simulink model "Controle_da_Haste"  (R2025b)
settings: Solver=ode4  StartTime=0.0  StopTime=inf  FixedStep=0.01  RelTol=1e-3  EnableMultiTasking=on
undefined symbols (not defined in the file): bits
libraries: stm32blockslib x7
settings Model: STM32="{\"I2CControllerWrite\":[{\"ID\":\"untitled:10\"},{\"ID\":\"untitled:31\"},{\"ID\":\"untitled:32\"},{\"ID\":\"untitled:33\"},{\"ID\":\"Controle_da_Haste:31\"},{\"ID\":\"Controle_da_Haste:32\"},{\"ID\":\"Controle_da_Haste:33\"},{\"ID\":\"Controle_da_Haste:152\"},{\"ID\":\"Controle_da_Haste:153\"},{\"ID\":\"Controle_da_Haste:154\"},{\"ID\":\"Controle_da_Haste:10\"}],\"I2CControllerRead\":[{\"ID\":\"untitled:43\"},{\"ID\":\"Controle_da_Haste:43\"},{\"ID\":\"Controle_da_Haste:163\"}],\"EncoderBlock\":[{\"ID\":\"untitled:57\"},{\"ID\":\"Controle_da_Haste:57\"}],\"SPIControllerTransfer\":{\"ID\":\"Controle_da_Haste:81\"}}"  Creator=IEE-S  LastModifiedBy=IEE-S
settings OptimizationCC: EnhancedBackFolding=on  PassReuseOutputArgsAs=Individual arguments  ZeroExternalMemoryAtStartup=off  ZeroInternalMemoryAtStartup=off  MaxStackSize=512  OptimizeBlockOrder=speed  DifferentSizesBufferReuse=on  OptimizationCustomize=off  EfficientTunableParamExpr=on
settings DebuggingCC: ParameterTunabilityLossMsg=error
settings HardwareCC: ProdBitPerPointer=32.0  ProdBitPerSizeT=32.0  ProdBitPerPtrDiffT=32.0  ProdLargestAtomicInteger=Long  ProdLargestAtomicFloat=Double  ProdWordSize=32.0  ProdLongLongMode=on  ProdHWDeviceType=ARM Compatible->ARM Cortex-M
settings SFSimCC: MATLABDynamicMemAlloc=off
settings RTWCC: SystemTargetFile=ert.tlc  HardwareBoard=STM32F4xx Based  TemplateMakefile=ert_default_tmf  Toolchain=GNU Tools for ARM Embedded Processors  Description=Embedded Coder
settings CodeAppCC: ForceParamTrailComments=on  IgnoreCustomStorageClasses=off  OperatorAnnotations=on  SimulinkDataObjDesc=on  SFDataObjDesc=on  InsertBlockDesc=on
settings ERTTargetCC: ExtModeTransport=3.0  ExtModeStaticAlloc=on  ExtModeStaticAllocSize=2048.0  ExtModeMexFile=ext_xcp  ExtModeIntrfLevel=Level2 - Open  InlinedParameterPlacement=Hierarchical  TargetLangStandard=C99 (ISO)  CodeReplacementLibrary=ARM Cortex-M

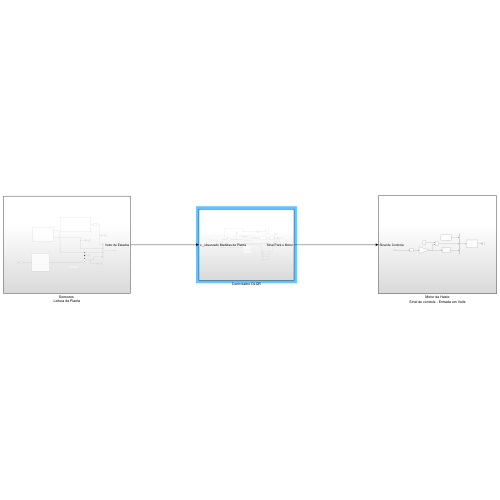
[thumbnail: Simulink's stored preview of the top-level diagram]
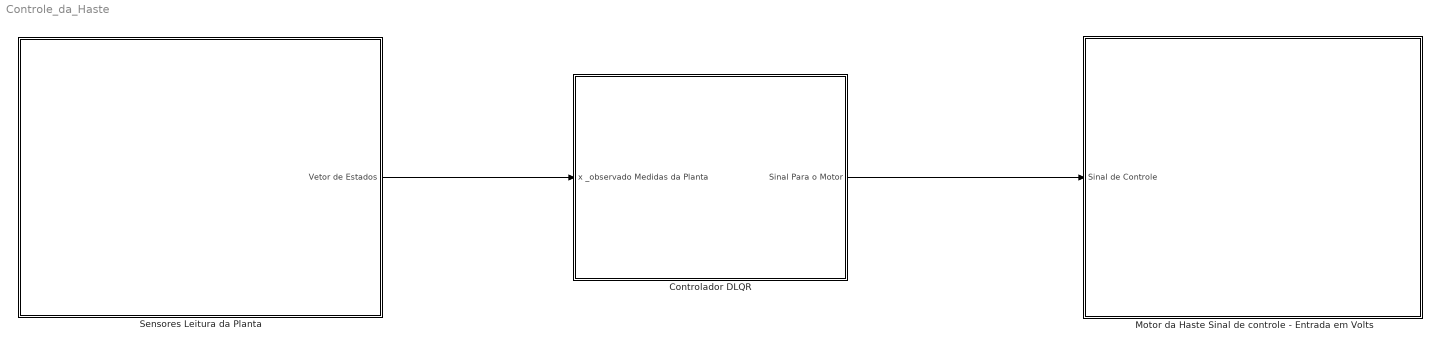
== system Controle_da_Haste ==
  Controlador DLQR : Subsystem
  Motor da Haste Sinal de controle - Entrada em Volts : Subsystem  Priority=6
  Sensores Leitura da Planta : Subsystem
  wires:
  Sensores Leitura da Planta/1(Vetor de Estados) -> Controlador DLQR/1(x _observado Medidas da Planta)
  Controlador DLQR/1(Sinal Para o Motor) -> Motor da Haste Sinal de controle - Entrada em Volts/1(Sinal de Controle)

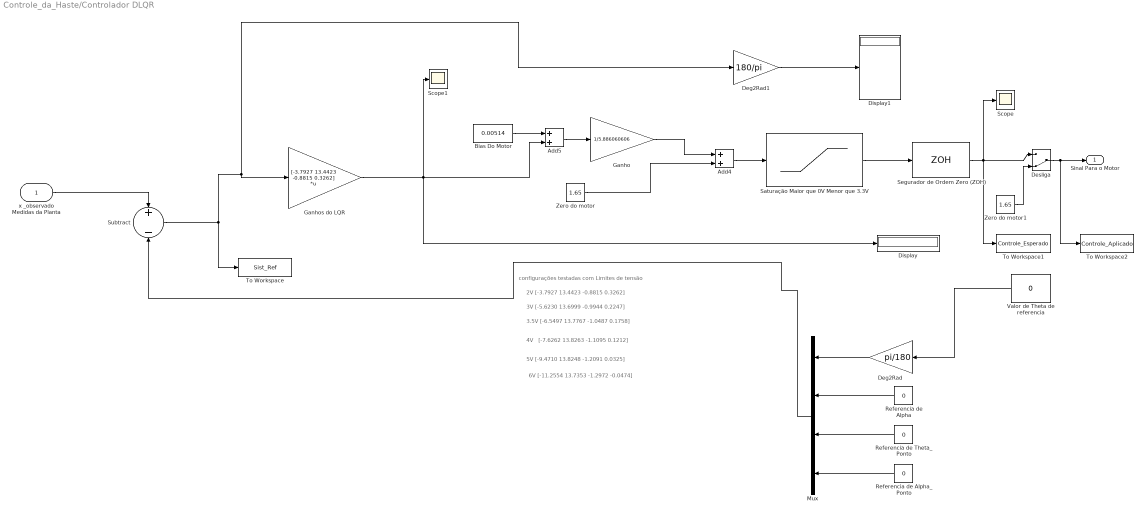
== system Controle_da_Haste/Controlador DLQR ==
  note: [-7.6262 13.8263 -1.1095 0.1212]
  note: 4V
  note: 3V [-5.6230 13.6999 -0.9944 0.2247]
  note: 2V [-3.7927 13.4423 -0.8815 0.3262]
  note: configurações testadas com Limites de tensão
  note: 3.5V [-6.5497 13.7767 -1.0487 0.1758]
  note: 5V [-9.4710 13.8248 -1.2091 0.0325]
  note: 6V [-11.2554 13.7353 -1.2972 -0.0474]
  x _observado Medidas da Planta : Inport
  Add4 : Sum
  Add5 : Sum
  Bias Do Motor : Constant  Value=0.00514
  Deg2Rad : Gain  Gain=pi/180
  Deg2Rad1 : Gain  Gain=180/pi
  Desliga : ManualSwitch  CurrentSetting=0
  Display : Display
  Display1 : Display
  Ganho : Gain  Gain=1/5.886060606
  Ganhos do LQR : Gain  Gain="[-3.7927  13.4423    -0.8815   0.3262]"  Multiplication=Matrix(K*u) (u vector)
  Mux : Mux
  Referencia de Alpha : Constant  Value=0
  Referencia de Alpha_Ponto : Constant  Value=0
  Referencia de Theta_Ponto : Constant  Value=0
  Saturação Maior que 0V Menor que 3.3V : Saturate  UpperLimit=3.3  LowerLimit=0
  Scope : Scope
      settings: ActiveDisplayYMinimum=1.3696990193816192  ActiveDisplayYMaximum=1.8844669389329192  DataLoggingVariableName=ScopeData4
  Scope1 : Scope
      settings: ActiveDisplayYMinimum=-26.689119690198989  ActiveDisplayYMaximum=29.989428485909986  DataLoggingVariableName=ScopeData5
  Segurador de Ordem Zero (ZOH) : ZeroOrderHold  SampleTime=-1
  Subtract : Sum  Inputs=+-
  To Workspace : ToWorkspace  VariableName=Sist_Ref  SaveFormat=Timeseries  SampleTime=-1
  To Workspace1 : ToWorkspace  VariableName=Controle_Esperado  SaveFormat=Timeseries  SampleTime=-1
  To Workspace2 : ToWorkspace  VariableName=Controle_Aplicado  SaveFormat=Timeseries  SampleTime=-1
  Valor de Theta de referencia : Constant  Value=0
  Zero do motor : Constant  Value=1.65
  Zero do motor1 : Constant  Value=1.65
  Sinal Para o Motor : Outport
  wires:
  x _observado Medidas da Planta/1 -> Subtract/1
  Bias Do Motor/1 -> Add5/1
  Ganho/1 -> Add4/1
  Zero do motor/1 -> Add4/2
  Add4/1 -> Saturação Maior que 0V Menor que 3.3V/1
  Add5/1 -> Ganho/1
  Ganhos do LQR/1 -> Scope1/1, Add5/2, Display/1
  Saturação Maior que 0V Menor que 3.3V/1 -> Segurador de Ordem Zero (ZOH)/1
  Subtract/1 -> To Workspace/1, Deg2Rad1/1, Ganhos do LQR/1
  Segurador de Ordem Zero (ZOH)/1 -> Scope/1, Desliga/1, To Workspace1/1
  Deg2Rad/1 -> Mux/1
  Referencia de Theta_Ponto/1 -> Mux/3
  Referencia de Alpha/1 -> Mux/2
  Referencia de Alpha_Ponto/1 -> Mux/4
  Mux/1 -> Subtract/2
  Desliga/1 -> To Workspace2/1, Sinal Para o Motor/1
  Zero do motor1/1 -> Desliga/2
  Valor de Theta de referencia/1 -> Deg2Rad/1
  Deg2Rad1/1 -> Display1/1

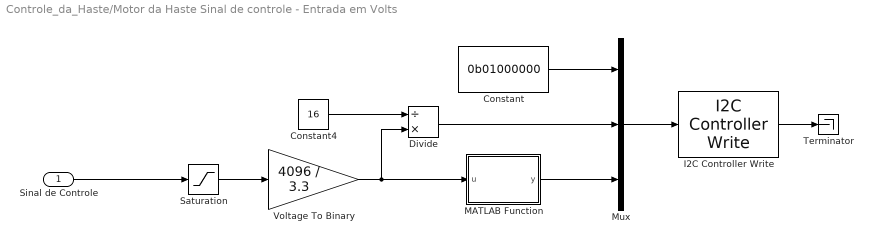
== system Controle_da_Haste/Motor da Haste Sinal de controle - Entrada em Volts ==
  Sinal de Controle : Inport
  Constant : Constant  Value=0b01000000  OutDataTypeStr=uint8
  Constant4 : Constant  Value=16
  Divide : Product  Inputs=/*  OutDataTypeStr=uint8
  I2C Controller Write : stm32blockslib/I2C Controller Write  I2CModule=I2C1  Mode=Controller  AddressingMode=7-bits  PeripheralByteOrder=BigEndian  OwnPeripheralAddress=uint8(170)  PeripheralAddressVia=Dialog  PeripheralAddress=0x60  RegisterAddressMode=off  RegisterAddressVia=Dialog  RegisterAddress=1  RepeatedStart=off  NoAck=off  OutputStatus=on  BlockMode=Transmit  DataType=uint8  DataLength=1  Timeout=0.001  SampleTime=-1
      settings: LibrarySourceBlock=stm32f4xxblockslib/I2C Controller Write
  MATLAB Function : MATLAB Function  TreatAsAtomicUnit=on
  Mux : Mux  Inputs=3
  Saturation : Saturate  UpperLimit=3.3  LowerLimit=0  OutDataTypeStr=Inherit: Inherit via back propagation
  Terminator : Terminator
  Voltage To Binary : Gain  Gain=4096 / 3.3  ParamDataTypeStr=uint16
  wires:
  Voltage To Binary/1 -> Divide/2, MATLAB Function/1(u)
  Constant4/1 -> Divide/1
  Constant/1 -> Mux/1
  Divide/1 -> Mux/2
  I2C Controller Write/1 -> Terminator/1
  MATLAB Function/1(y) -> Mux/3
  Saturation/1 -> Voltage To Binary/1
  Mux/1 -> I2C Controller Write/1
  Sinal de Controle/1 -> Saturation/1

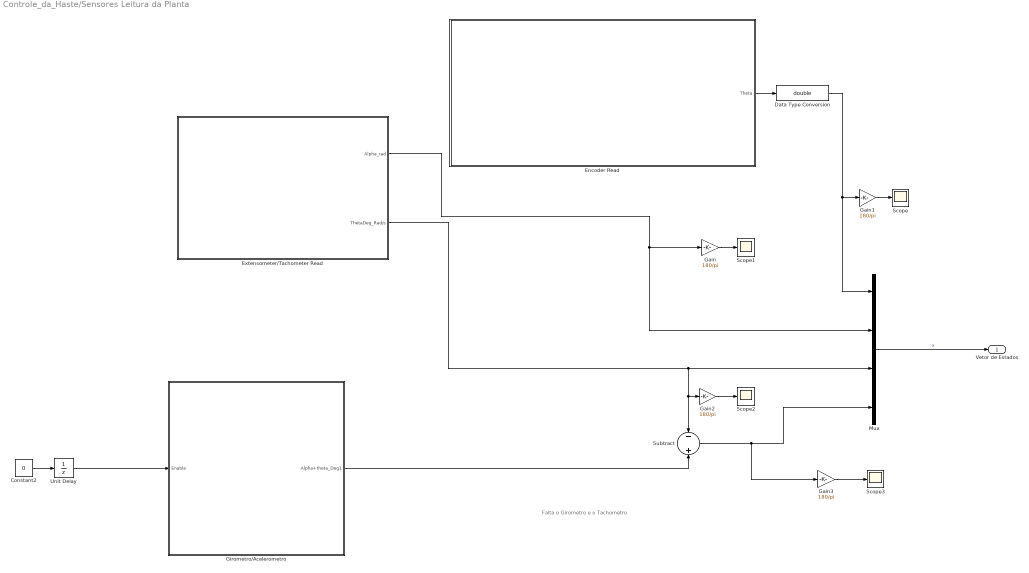
== system Controle_da_Haste/Sensores Leitura da Planta ==
  note: Falta o Girometro e o Tachometro
  Constant2 : Constant  Value=0
  Data Type Conversion : DataTypeConversion  OutDataTypeStr=double  RndMeth=Round  SaturateOnIntegerOverflow=off
  Encoder Read : Subsystem  Priority=3
  Extensometer/Tachometer Read : Subsystem  Priority=4
  Gain{,1..3} (4 alike) : Gain  Gain=180/pi
  Girometro/Acelerometro : Subsystem  Priority=1
  Mux : Mux
  Scope{,1..3} (4 alike) : Scope
      Scope settings: ActiveDisplayYMinimum=-37.614862788092672  ActiveDisplayYMaximum=73.168879201509782
      Scope1 settings: ActiveDisplayYMinimum=-4.0610934597852637  ActiveDisplayYMaximum=0.45969850920646227
      Scope2 settings: ActiveDisplayYMinimum=-2.80662625539894  ActiveDisplayYMaximum=8.42656069865145  DataLoggingVariableName=ScopeData2
      Scope3 settings: ActiveDisplayYMinimum=-35.050597654455132  ActiveDisplayYMaximum=20.146961930229978  DataLoggingVariableName=ScopeData3
  Subtract : Sum  Inputs=-+
  Unit Delay : UnitDelay  InitialCondition=1  SampleTime=-1  HasFrameUpgradeWarning=on
  Vetor de Estados : Outport
  wires:
  Mux/1 -> Vetor de Estados/1  "x"
  Extensometer/Tachometer Read/2(ThetaDeg_Rad/s) -> Gain2/1, Subtract/1, Mux/3
  Encoder Read/1(Theta) -> Data Type Conversion/1
  Subtract/1 -> Mux/4, Gain3/1
  Girometro/Acelerometro/1(Alpha+theta_Deg1) -> Subtract/2
  Unit Delay/1 -> Girometro/Acelerometro/1(Enable)
  Constant2/1 -> Unit Delay/1
  Extensometer/Tachometer Read/1(Alpha_rad) -> Mux/2, Gain/1
  Data Type Conversion/1 -> Gain1/1, Mux/1
  Gain/1 -> Scope1/1
  Gain1/1 -> Scope/1
  Gain2/1 -> Scope2/1
  Gain3/1 -> Scope3/1

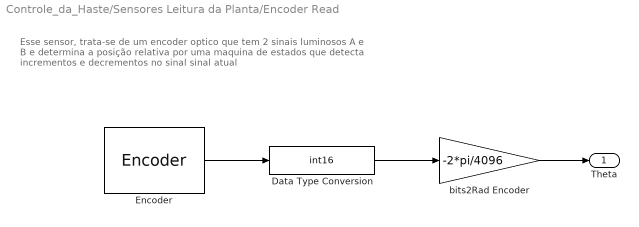
== system Controle_da_Haste/Sensores Leitura da Planta/Encoder Read ==
  note: Esse sensor, trata-se de um encoder optico que tem 2 sinais luminosos A e B e determina a posição relativa por uma maquina de estados que detecta incrementos e decrementos no sinal sinal atual
  Data Type Conversion : DataTypeConversion  OutDataTypeStr=int16  RndMeth=Round  SaturateOnIntegerOverflow=off
  Encoder : stm32blockslib/Encoder  TimerModule=TIM4  EnableResetInput=off  OutputDirection=off  SampleTime=-1
      settings: LibrarySourceBlock=stm32f4xxblockslib/Encoder
  bits2Rad Encoder : Gain  Gain=-2*pi/4096
  Theta : Outport
  wires:
  Encoder/1 -> Data Type Conversion/1
  Data Type Conversion/1 -> bits2Rad Encoder/1
  bits2Rad Encoder/1 -> Theta/1

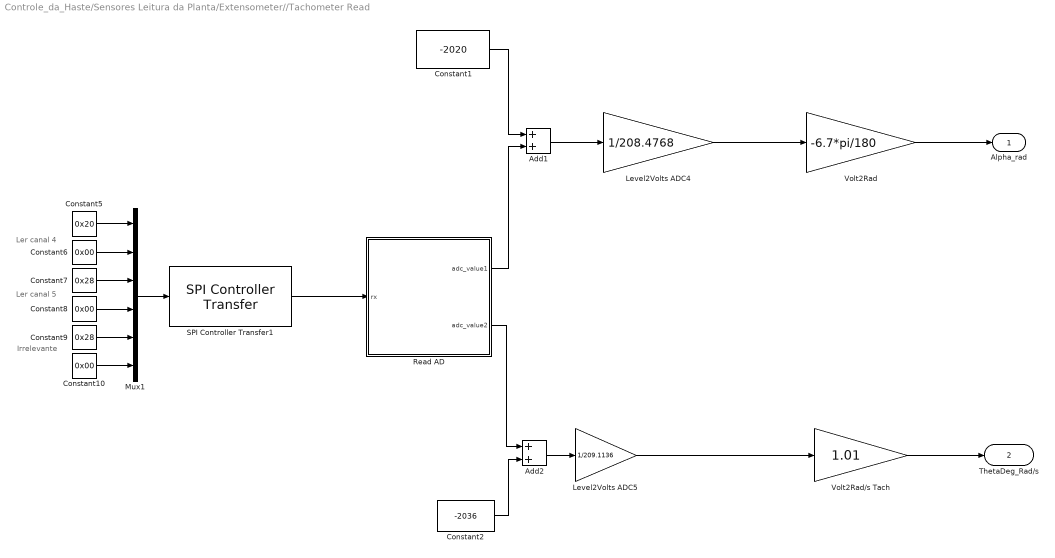
== system Controle_da_Haste/Sensores Leitura da Planta/Extensometer//Tachometer Read ==
  note: Irrelevante
  note: Ler canal 5
  note: Ler canal 4
  Add1 : Sum
  Add2 : Sum
  Constant1 : Constant  Value=-2020
  Constant10 : Constant  Value=0x00  OutDataTypeStr=uint8
  Constant2 : Constant  Value=-2036
  Constant5 : Constant  Value=0x20  OutDataTypeStr=uint8
  Constant6 : Constant  Value=0x00  OutDataTypeStr=uint8
  Constant7 : Constant  Value=0x28  OutDataTypeStr=uint8
  Constant8 : Constant  Value=0x00  OutDataTypeStr=uint8
  Constant9 : Constant  Value=0x28  OutDataTypeStr=uint8
  Level2Volts ADC4 : Gain  Gain=1/208.4768
  Level2Volts ADC5 : Gain  Gain=1/209.1136
  Mux1 : Mux  Inputs=6
  Read AD : MATLAB Function  TreatAsAtomicUnit=on
  SPI Controller Transfer1 : stm32blockslib/SPI Controller Transfer  SPIModuleSelect=SPI2  ClockPolarity=Low  ClockPhase=1 Edge  SPIModule=uint32(0)  Mode=Master  BusSpeed=uint32(1000000)  FirstBitToTransfer=Most significant bit (MSB)  ClockMode=0  BlockFunction=Transfer  EnableRegisterAddress=off  RegisterAddress=0  OutputDataType=uint8  OutputDataLength=1  OutputStatus=off  BlockingMode=on  Timeout=1  DataBits=8  UseCustomSSPin=Explicit GPIO calls  ActiveLowSSPin=Active low  Port_Select=GPIOA  Pin=4
      settings: LibrarySourceBlock=stm32f4xxblockslib/SPI Controller Transfer
  Volt2Rad : Gain  Gain=-6.7*pi/180
  Volt2Rad/s Tach : Gain  Gain=1.01
  Alpha_rad : Outport
  ThetaDeg_Rad/s : Outport  Port=2
  wires:
  Constant8/1 -> Mux1/4
  Constant7/1 -> Mux1/3
  Constant5/1 -> Mux1/1
  Mux1/1 -> SPI Controller Transfer1/1
  SPI Controller Transfer1/1 -> Read AD/1(rx)
  Constant6/1 -> Mux1/2
  Constant10/1 -> Mux1/6
  Constant9/1 -> Mux1/5
  Level2Volts ADC5/1 -> Volt2Rad/s Tach/1
  Level2Volts ADC4/1 -> Volt2Rad/1
  Volt2Rad/s Tach/1 -> ThetaDeg_Rad/s/1
  Volt2Rad/1 -> Alpha_rad/1
  Add1/1 -> Level2Volts ADC4/1
  Read AD/1(adc_value1) -> Add1/2
  Constant1/1 -> Add1/1
  Add2/1 -> Level2Volts ADC5/1
  Read AD/2(adc_value2) -> Add2/1
  Constant2/1 -> Add2/2

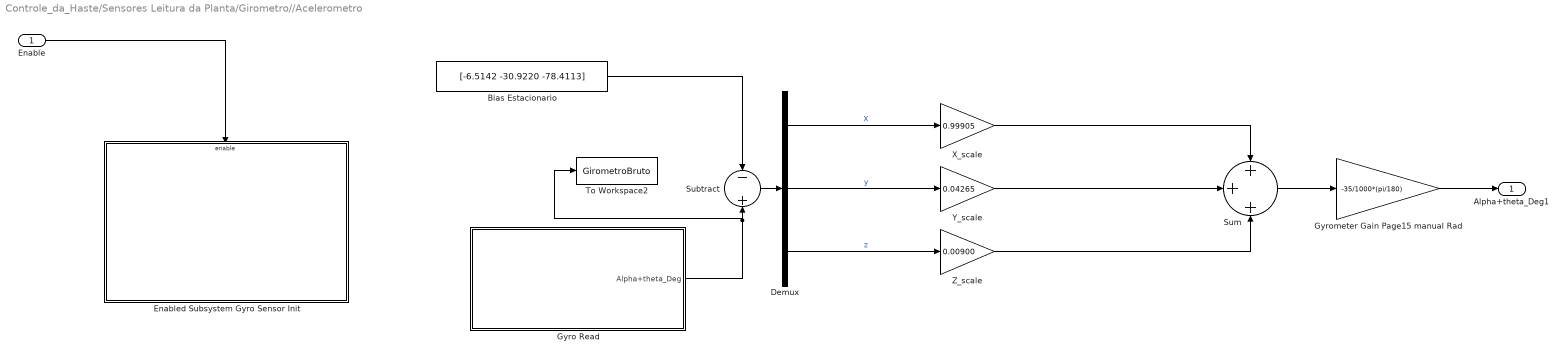
== system Controle_da_Haste/Sensores Leitura da Planta/Girometro//Acelerometro ==
  Enable : Inport
  Bias Estacionario : Constant  Value=[-6.5142 -30.9220 -78.4113]
  Demux : Demux  Outputs=3
  Enabled Subsystem Gyro Sensor Init : Subsystem  Priority=1  TreatAsAtomicUnit=on
  Gyro Read : Subsystem  Priority=2
  Gyrometer Gain Page15 manual Rad : Gain  Gain=-35/1000*(pi/180)
  Subtract : Sum  Inputs=-+
  Sum : Sum  Inputs=+++
  To Workspace2 : ToWorkspace  VariableName=GirometroBruto  SaveFormat=Timeseries  SampleTime=-1
  X_scale : Gain  Gain=0.99905
  Y_scale : Gain  Gain=0.04265
  Z_scale : Gain  Gain=0.00900
  Alpha+theta_Deg1 : Outport
  wires:
  Enable/1 -> Enabled Subsystem Gyro Sensor Init/Enable
  Gyro Read/1(Alpha+theta_Deg) -> To Workspace2/1, Subtract/2
  Demux/3 -> Z_scale/1  "z"
  Demux/1 -> X_scale/1  "X"
  Gyrometer Gain Page15 manual Rad/1 -> Alpha+theta_Deg1/1
  Y_scale/1 -> Sum/2
  Sum/1 -> Gyrometer Gain Page15 manual Rad/1
  Z_scale/1 -> Sum/3
  X_scale/1 -> Sum/1
  Demux/2 -> Y_scale/1  "y"
  Bias Estacionario/1 -> Subtract/1
  Subtract/1 -> Demux/1

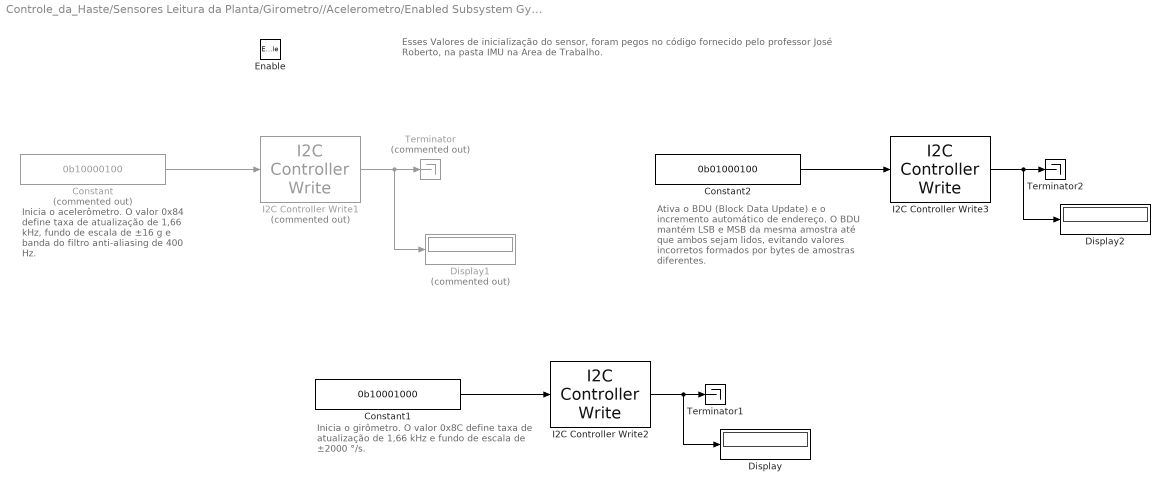
== system Controle_da_Haste/Sensores Leitura da Planta/Girometro//Acelerometro/Enabled Subsystem Gyro Sensor Init ==
  note: Inicia o acelerômetro. O valor 0x84 define taxa de atualização
      | de 1,66 kHz, fundo de escala de ±16 g e banda do filtro anti-aliasing de 400 Hz.
  note: Inicia o girômetro. O valor 0x8C define taxa de atualização
      | de 1,66 kHz e fundo de escala de ±2000 °/s.
  note: Ativa o BDU (Block Data Update) e o incremento automático de endereço.
      | O BDU mantém LSB e MSB da mesma amostra até que ambos sejam lidos,
      | evitando valores incorretos formados por bytes de amostras diferentes.
  note: Esses Valores de inicialização do sensor, foram pegos no código fornecido pelo professor José Roberto, na pasta IMU na Area de Trabalho.
  Enable : EnablePort
  Constant : Constant  Commented=on  Value=0b10000100
  Constant1 : Constant  Value=0b10001000
  Constant2 : Constant  Value=0b01000100
  Display : Display
  Display1 : Display  Commented=on
  Display2 : Display
  I2C Controller Write1 : stm32blockslib/I2C Controller Write  Commented=on  I2CModule=I2C1  Mode=Controller  AddressingMode=7-bits  PeripheralByteOrder=BigEndian  OwnPeripheralAddress=uint8(170)  PeripheralAddressVia=Dialog  PeripheralAddress=0b1101010  RegisterAddressMode=on  RegisterAddressVia=Dialog  RegisterAddress=0x10  RepeatedStart=off  NoAck=off  OutputStatus=on  BlockMode=Transmit  DataType=uint8  DataLength=1  Timeout=0.001  SampleTime=-1
      settings: LibrarySourceBlock=stm32f4xxblockslib/I2C Controller Write
  I2C Controller Write2 : stm32blockslib/I2C Controller Write  I2CModule=I2C1  Mode=Controller  AddressingMode=7-bits  PeripheralByteOrder=BigEndian  OwnPeripheralAddress=uint8(170)  PeripheralAddressVia=Dialog  PeripheralAddress=0b1101010  RegisterAddressMode=on  RegisterAddressVia=Dialog  RegisterAddress=0x11  RepeatedStart=off  NoAck=off  OutputStatus=on  BlockMode=Transmit  DataType=uint8  DataLength=1  Timeout=0.001  SampleTime=-1
      settings: LibrarySourceBlock=stm32f4xxblockslib/I2C Controller Write
  I2C Controller Write3 : stm32blockslib/I2C Controller Write  I2CModule=I2C1  Mode=Controller  AddressingMode=7-bits  PeripheralByteOrder=BigEndian  OwnPeripheralAddress=uint8(170)  PeripheralAddressVia=Dialog  PeripheralAddress=0x6A  RegisterAddressMode=on  RegisterAddressVia=Dialog  RegisterAddress=0x12  RepeatedStart=off  NoAck=off  OutputStatus=on  BlockMode=Transmit  DataType=uint8  DataLength=1  Timeout=0.001  SampleTime=-1
      settings: LibrarySourceBlock=stm32f4xxblockslib/I2C Controller Write
  Terminator : Terminator  Commented=on
  Terminator1 : Terminator
  Terminator2 : Terminator
  wires:
  Constant/1 -> I2C Controller Write1/1
  I2C Controller Write1/1 -> Display1/1, Terminator/1
  I2C Controller Write2/1 -> Display/1, Terminator1/1
  Constant1/1 -> I2C Controller Write2/1
  Constant2/1 -> I2C Controller Write3/1
  I2C Controller Write3/1 -> Terminator2/1, Display2/1

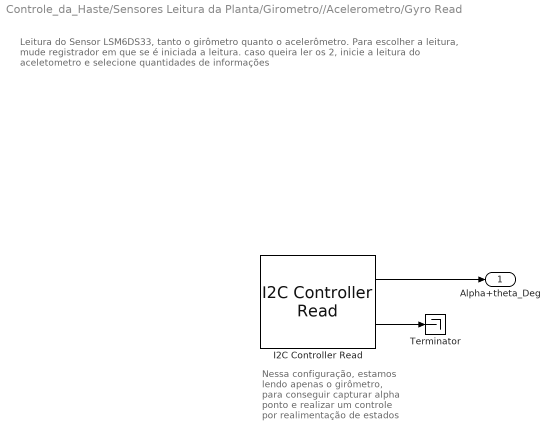
== system Controle_da_Haste/Sensores Leitura da Planta/Girometro//Acelerometro/Gyro Read ==
  note: Nessa configuração, estamos lendo apenas o girômetro, para conseguir capturar alpha ponto e realizar um controle por realimentação de estados
  note: Leitura do Sensor LSM6DS33, tanto o girômetro quanto o acelerômetro. Para escolher a leitura, mude registrador em que se é iniciada a leitura. caso queira ler os 2, inicie a leitura do aceletometro e selecione quantidades de informações
  I2C Controller Read : stm32blockslib/I2C Controller Read  I2CModule=I2C1  Mode=Controller  AddressingMode=7-bits  PeripheralByteOrder=LittleEndian  OwnPeripheralAddress=uint8(170)  PeripheralAddressVia=Dialog  PeripheralAddress=0b1101010  RegisterAddressMode=on  RegisterAddressVia=Dialog  RegisterAddress=0x22  RepeatedStart=off  NoAck=off  OutputStatus=on  BlockMode=Receive  DataType=int16  DataLength=3  Timeout=0.010  SampleTime=-1
      settings: LibrarySourceBlock=stm32f4xxblockslib/I2C Controller Read
  Terminator : Terminator
  Alpha+theta_Deg : Outport
  wires:
  I2C Controller Read/1 -> Alpha+theta_Deg/1
  I2C Controller Read/2 -> Terminator/1

== matlab function Controle_da_Haste/Sensores Leitura da Planta/Extensometer//Tachometer Read/Read AD ==
  data: rx input; adc_value1 output; adc_value2 output
function [adc_value1, adc_value2] = decode_adc120(rx)

% Valor 1: bytes 3 e 4
raw1 = bitor(bitshift(uint16(rx(3)),8), uint16(rx(4)));
adc_value1 = bitand(raw1, hex2dec('0FFF'));

% Valor 2: bytes 5 e 6
raw2 = bitor(bitshift(uint16(rx(5)),8), uint16(rx(6)));
adc_value2 = bitand(raw2, hex2dec('0FFF'));

end

== matlab function Controle_da_Haste/Motor da Haste Sinal de controle - Entrada em Volts/MATLAB Function ==
  data: u input; y output
function y = fcn(u)

y = bitshift(bitand(u, uint8(15)), 4);
